simulink model "lr4_v20_task1_d0"  (R2023a)
settings: Solver=ode45  StartTime=5  StopTime=7  RelTol=1e-9  AbsTol=1e-11
InitFcn:
  | h=0.01; a=18; p=2; q=4;
settings Model: Creator=theju  LastModifiedBy=theju

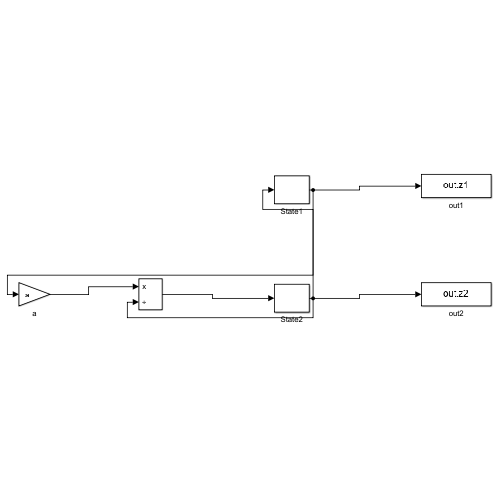
[thumbnail: Simulink's stored preview of the top-level diagram]
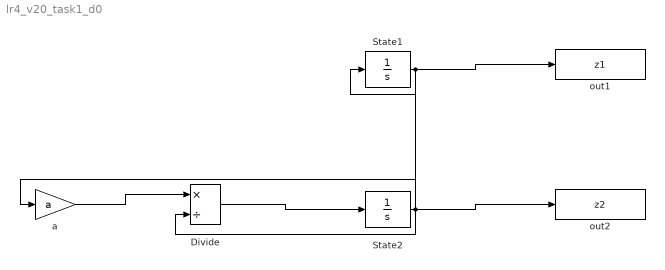
== system lr4_v20_task1_d0 ==
  Divide : Product  Inputs=*/
  State1 : Integrator  InitialCondition=1
  State2 : Integrator  InitialCondition=3
  a : Gain  Gain=a
  out1 : ToWorkspace  VariableName=z1  SaveFormat=Timeseries  SampleTime=-1
  out2 : ToWorkspace  VariableName=z2  SaveFormat=Timeseries  SampleTime=-1
  wires:
  State1/1 -> out1/1, a/1
  State2/1 -> out2/1, State1/1, Divide/2
  a/1 -> Divide/1
  Divide/1 -> State2/1
